simulink model "s_b16a4x32kf"  (R2018a)
settings: Solver=VariableStepDiscrete  StartTime=0.0  StopTime=1000  RelTol=1e-3
undefined symbols (not defined in the file): fft_stages, n_bits_ants, n_bits_xengs
libraries: xbsIndex_r4 x23740, casper_library_misc x48, casper_library_delays x8, xps_library x4, casper_library_scopes x1
(part 48 of 219)

== system s_b16a4x32kf/sys0/xeng/baseline_tap7 ==
  a_del : Inport
  a_ndel : Inport  Port=2
  a_end : Inport  Port=3
  acc_in : Inport  Port=4
  valid_in : Inport  Port=5
  rst : Inport  Port=6
  sync1 : Inport  Port=7
  Constant : xbsIndex_r4/Constant  const=ant_sep * acc_len  gui_display_data_type=Fixed-point  arith_type=Unsigned  n_bits=ant_bits + bit_growth  bin_pt=0  preci_type=Single  exp_width=8  frac_width=24  explicit_period=on  period=1  equ=P=C  opselect=C  inp2=PCIN>>17  opr=+  inp1=P  carry=CIN  dbl_ovrd=off  block_type=constant
      settings: block_version=9.1.01
  Convert : xbsIndex_r4/Convert  gui_display_data_type=Fixed-point  arith_type=Unsigned  n_bits=1  bin_pt=0  float_type=Single  exp_bits=8  fraction_bits=24  quantization=Truncate  overflow=Wrap  en=off  latency=0  pipeline=off  dbl_ovrd=off  block_type=convert
      settings: xl_area=[0, 0, 0, 0, 0, 0, 0]
  Counter : xbsIndex_r4/Counter  cnt_type=Count Limited  cnt_to=n_ants * acc_len - 1  operation=Up  start_count=0  cnt_by_val=1  arith_type=Unsigned  n_bits=ant_bits + bit_growth  bin_pt=0  load_pin=off  rst=on  en=off  explicit_period=off  period=1  use_behavioral_HDL=off  implementation=Fabric  use_rpm=on  dbl_ovrd=off  block_type=counter
      settings: xl_area=[0, 0, 0, 0, 0, 0, 0]  block_version=9.1.01
  Delay{1,3,7..8} (4 alike) : xbsIndex_r4/Delay  rst=off  infoeditControl=Selection of Reset will increase slice count due to use of real FFs and instead of SRLs  en=off  latency=1  reg_retiming=on  dbl_ovrd=off  block_type=delay
      settings: xl_area=[0, 0, 0, 0, 0, 0, 0]  block_version=9.1.01
  Mux : xbsIndex_r4/Mux  inputs=2  en=off  latency=1  precision=Full  arith_type="Signed  (2's comp)"  n_bits=8  bin_pt=2  quantization=Truncate  overflow=Wrap  dbl_ovrd=off  block_type=mux
      settings: xl_area=[0, 0, 0, 0, 0, 0, 0]  block_version=9.1.01
  Relational : xbsIndex_r4/Relational  mode=a<b  op_type=Bool  en=off  latency=0  dbl_ovrd=off  block_type=relational
      settings: xl_area=[0, 0, 0, 0, 0, 0, 0]  block_version=9.1.01
  delay : Subsystem  AncestorBlock=casper_library_delays/delay_bram  mask(delay_bram){DelayLen=acc_len, bram_latency=bram_latency, use_dsp48=off, async=off}
      mask prompts: DelayLen "Delay By:"; bram_latency "BRAM Latency"; use_dsp48 "Use DSP48"; async "asynchronous operation"
      mask help: A delay block that uses BRAM for its storage.
      mask init:
      | delay_bram_init(gcb, ...
      |     'DelayLen', DelayLen, ...
      |     'bram_latency', bram_latency, ...
      |     'use_dsp48', use_dsp48, ...
      |     'async', async);
      mask Help: eval('xlWeb(''http://casper.berkeley.edu/wiki/Delay_bram'')')
  dual_pol_cmac : Subsystem  AncestorBlock=casper_library_correlator/dual_pol_cmac  mask{acc_len=256, n_bits_in=8, bin_pt_in=7, mult_latency=4, add_latency=3, multiplier_implementation=embedded multiplier core}
      mask prompts: acc_len "Number of accumulations"; n_bits_in "Number of bits in"; bin_pt_in "Binary point in"; mult_latency "Multiplier latency"; add_latency "Adder latency"; multiplier_implementation "Multiplier implementation"
      mask init: same as s_b16a4x32kf/sys0/xeng/auto_tap/dual_pol_cmac
      mask TypeOptions multiplier_implementation: behavioral HDL | standard core | embedded multiplier core
  a_del_out : Outport
  a_ndel_out : Outport  Port=2
  a_end_out : Outport  Port=3
  acc_out : Outport  Port=4
  valid_out : Outport  Port=5
  rst_out : Outport  Port=6
  sync_out : Outport  Port=7
  wires:
  delay/1(dout) -> Delay3/1
  Mux/1 -> dual_pol_cmac/2(a2)
  Counter/1 -> Relational/1
  Constant/1 -> Relational/2
  Relational/1 -> Convert/1
  Convert/1 -> Mux/1
  rst/1 -> Delay1/1, Counter/1
  a_del/1 -> delay/1(din)
  dual_pol_cmac/1(acc_out) -> acc_out/1
  acc_in/1 -> dual_pol_cmac/3(acc_in)
  dual_pol_cmac/2(valid_out) -> valid_out/1
  valid_in/1 -> dual_pol_cmac/5(valid_in)
  a_ndel/1 -> Mux/2, Delay7/1
  a_end/1 -> Mux/3, Delay8/1
  Delay3/1 -> a_del_out/1, dual_pol_cmac/1(a1)
  Delay7/1 -> a_ndel_out/1
  Delay8/1 -> a_end_out/1
  Delay1/1 -> rst_out/1, dual_pol_cmac/4(sync)
  sync1/1 -> sync_out/1

== system s_b16a4x32kf/sys0/xeng/baseline_tap8 ==
  a_del : Inport
  a_ndel : Inport  Port=2
  a_end : Inport  Port=3
  acc_in : Inport  Port=4
  valid_in : Inport  Port=5
  rst : Inport  Port=6
  sync1 : Inport  Port=7
  Constant : xbsIndex_r4/Constant  const=ant_sep * acc_len  gui_display_data_type=Fixed-point  arith_type=Unsigned  n_bits=ant_bits + bit_growth  bin_pt=0  preci_type=Single  exp_width=8  frac_width=24  explicit_period=on  period=1  equ=P=C  opselect=C  inp2=PCIN>>17  opr=+  inp1=P  carry=CIN  dbl_ovrd=off  block_type=constant
      settings: block_version=9.1.01
  Convert : xbsIndex_r4/Convert  gui_display_data_type=Fixed-point  arith_type=Unsigned  n_bits=1  bin_pt=0  float_type=Single  exp_bits=8  fraction_bits=24  quantization=Truncate  overflow=Wrap  en=off  latency=0  pipeline=off  dbl_ovrd=off  block_type=convert
      settings: xl_area=[0, 0, 0, 0, 0, 0, 0]
  Counter : xbsIndex_r4/Counter  cnt_type=Count Limited  cnt_to=n_ants * acc_len - 1  operation=Up  start_count=0  cnt_by_val=1  arith_type=Unsigned  n_bits=ant_bits + bit_growth  bin_pt=0  load_pin=off  rst=on  en=off  explicit_period=off  period=1  use_behavioral_HDL=off  implementation=Fabric  use_rpm=on  dbl_ovrd=off  block_type=counter
      settings: xl_area=[0, 0, 0, 0, 0, 0, 0]  block_version=9.1.01
  Delay{1,3,7..8} (4 alike) : xbsIndex_r4/Delay  rst=off  infoeditControl=Selection of Reset will increase slice count due to use of real FFs and instead of SRLs  en=off  latency=1  reg_retiming=on  dbl_ovrd=off  block_type=delay
      settings: xl_area=[0, 0, 0, 0, 0, 0, 0]  block_version=9.1.01
  Mux : xbsIndex_r4/Mux  inputs=2  en=off  latency=1  precision=Full  arith_type="Signed  (2's comp)"  n_bits=8  bin_pt=2  quantization=Truncate  overflow=Wrap  dbl_ovrd=off  block_type=mux
      settings: xl_area=[0, 0, 0, 0, 0, 0, 0]  block_version=9.1.01
  Relational : xbsIndex_r4/Relational  mode=a<b  op_type=Bool  en=off  latency=0  dbl_ovrd=off  block_type=relational
      settings: xl_area=[0, 0, 0, 0, 0, 0, 0]  block_version=9.1.01
  delay : Subsystem  AncestorBlock=casper_library_delays/delay_bram  mask(delay_bram){DelayLen=acc_len, bram_latency=bram_latency, use_dsp48=off, async=off}
      mask prompts: DelayLen "Delay By:"; bram_latency "BRAM Latency"; use_dsp48 "Use DSP48"; async "asynchronous operation"
      mask help: A delay block that uses BRAM for its storage.
      mask init:
      | delay_bram_init(gcb, ...
      |     'DelayLen', DelayLen, ...
      |     'bram_latency', bram_latency, ...
      |     'use_dsp48', use_dsp48, ...
      |     'async', async);
      mask Help: eval('xlWeb(''http://casper.berkeley.edu/wiki/Delay_bram'')')
  dual_pol_cmac : Subsystem  AncestorBlock=casper_library_correlator/dual_pol_cmac  mask{acc_len=256, n_bits_in=8, bin_pt_in=7, mult_latency=4, add_latency=3, multiplier_implementation=embedded multiplier core}
      mask prompts: acc_len "Number of accumulations"; n_bits_in "Number of bits in"; bin_pt_in "Binary point in"; mult_latency "Multiplier latency"; add_latency "Adder latency"; multiplier_implementation "Multiplier implementation"
      mask init: same as s_b16a4x32kf/sys0/xeng/auto_tap/dual_pol_cmac
      mask TypeOptions multiplier_implementation: behavioral HDL | standard core | embedded multiplier core
  a_del_out : Outport
  a_ndel_out : Outport  Port=2
  a_end_out : Outport  Port=3
  acc_out : Outport  Port=4
  valid_out : Outport  Port=5
  rst_out : Outport  Port=6
  sync_out : Outport  Port=7
  wires:
  delay/1(dout) -> Delay3/1
  Mux/1 -> dual_pol_cmac/2(a2)
  Counter/1 -> Relational/1
  Constant/1 -> Relational/2
  Relational/1 -> Convert/1
  Convert/1 -> Mux/1
  rst/1 -> Delay1/1, Counter/1
  a_del/1 -> delay/1(din)
  dual_pol_cmac/1(acc_out) -> acc_out/1
  acc_in/1 -> dual_pol_cmac/3(acc_in)
  dual_pol_cmac/2(valid_out) -> valid_out/1
  valid_in/1 -> dual_pol_cmac/5(valid_in)
  a_ndel/1 -> Mux/2, Delay7/1
  a_end/1 -> Mux/3, Delay8/1
  Delay3/1 -> a_del_out/1, dual_pol_cmac/1(a1)
  Delay7/1 -> a_ndel_out/1
  Delay8/1 -> a_end_out/1
  Delay1/1 -> rst_out/1, dual_pol_cmac/4(sync)
  sync1/1 -> sync_out/1

== system s_b16a4x32kf/sys0/xeng/sample_and_hold1 ==
  sync : Inport
  in : Inport  Port=2
  Constant3 : xbsIndex_r4/Constant  const=period-1  gui_display_data_type=Fixed-point  arith_type=Unsigned  n_bits=ceil(log2(period))  bin_pt=0  preci_type=Single  exp_width=8  frac_width=24  explicit_period=on  period=1  equ=P=C  opselect=C  inp2=PCIN>>17  opr=+  inp1=P  carry=CIN  dbl_ovrd=off  block_type=constant
  Counter4 : xbsIndex_r4/Counter  cnt_type=Free Running  cnt_to=Inf  operation=Up  start_count=0  cnt_by_val=1  arith_type=Unsigned  n_bits=ceil(log2(period))  bin_pt=0  load_pin=off  rst=on  en=off  explicit_period=on  period=1  use_behavioral_HDL=off  implementation=Fabric  use_rpm=on  dbl_ovrd=off  block_type=counter
      settings: xl_area=[0, 0, 0, 0, 0, 0, 0]
  Delay10 : xbsIndex_r4/Delay  rst=off  infoeditControl=Selection of Reset will increase slice count due to use of real FFs and instead of SRLs  en=off  latency=1  reg_retiming=on  dbl_ovrd=off  block_type=delay
      settings: xl_area=[0, 0, 0, 0, 0, 0, 0]
  Logical : xbsIndex_r4/Logical  logical_function=OR  inputs=2  en=off  latency=0  precision=Full  arith_type=Unsigned  n_bits=16  bin_pt=0  align_bp=on  dbl_ovrd=off  block_type=logical
  Register : xbsIndex_r4/Register  init=0  rst=off  en=on  dbl_ovrd=off  block_type=register
  Relational : xbsIndex_r4/Relational  mode=a>=b  op_type=Bool  en=off  latency=0  dbl_ovrd=off  block_type=relational
      settings: xl_area=[0, 0, 0, 0, 0, 0, 0]  block_version=10.1.3
  out : Outport
  wires:
  Relational/1 -> Logical/1
  Constant3/1 -> Relational/2
  Counter4/1 -> Relational/1
  Logical/1 -> Counter4/1, Delay10/1
  sync/1 -> Logical/2
  Register/1 -> out/1
  in/1 -> Register/1
  Delay10/1 -> Register/2

== system s_b16a4x32kf/sys0/xeng/sample_and_hold2 ==
  sync : Inport
  in : Inport  Port=2
  Constant3 : xbsIndex_r4/Constant  const=period-1  gui_display_data_type=Fixed-point  arith_type=Unsigned  n_bits=ceil(log2(period))  bin_pt=0  preci_type=Single  exp_width=8  frac_width=24  explicit_period=on  period=1  equ=P=C  opselect=C  inp2=PCIN>>17  opr=+  inp1=P  carry=CIN  dbl_ovrd=off  block_type=constant
  Counter4 : xbsIndex_r4/Counter  cnt_type=Free Running  cnt_to=Inf  operation=Up  start_count=0  cnt_by_val=1  arith_type=Unsigned  n_bits=ceil(log2(period))  bin_pt=0  load_pin=off  rst=on  en=off  explicit_period=on  period=1  use_behavioral_HDL=off  implementation=Fabric  use_rpm=on  dbl_ovrd=off  block_type=counter
      settings: xl_area=[0, 0, 0, 0, 0, 0, 0]
  Delay10 : xbsIndex_r4/Delay  rst=off  infoeditControl=Selection of Reset will increase slice count due to use of real FFs and instead of SRLs  en=off  latency=1  reg_retiming=on  dbl_ovrd=off  block_type=delay
      settings: xl_area=[0, 0, 0, 0, 0, 0, 0]
  Logical : xbsIndex_r4/Logical  logical_function=OR  inputs=2  en=off  latency=0  precision=Full  arith_type=Unsigned  n_bits=16  bin_pt=0  align_bp=on  dbl_ovrd=off  block_type=logical
  Register : xbsIndex_r4/Register  init=0  rst=off  en=on  dbl_ovrd=off  block_type=register
  Relational : xbsIndex_r4/Relational  mode=a>=b  op_type=Bool  en=off  latency=0  dbl_ovrd=off  block_type=relational
      settings: xl_area=[0, 0, 0, 0, 0, 0, 0]  block_version=10.1.3
  out : Outport
  wires:
  Relational/1 -> Logical/1
  Constant3/1 -> Relational/2
  Counter4/1 -> Relational/1
  Logical/1 -> Counter4/1, Delay10/1
  sync/1 -> Logical/2
  Register/1 -> out/1
  in/1 -> Register/1
  Delay10/1 -> Register/2

== system s_b16a4x32kf/sys0/xeng/sample_and_hold3 ==
  sync : Inport
  in : Inport  Port=2
  Constant3 : xbsIndex_r4/Constant  const=period-1  gui_display_data_type=Fixed-point  arith_type=Unsigned  n_bits=ceil(log2(period))  bin_pt=0  preci_type=Single  exp_width=8  frac_width=24  explicit_period=on  period=1  equ=P=C  opselect=C  inp2=PCIN>>17  opr=+  inp1=P  carry=CIN  dbl_ovrd=off  block_type=constant
  Counter4 : xbsIndex_r4/Counter  cnt_type=Free Running  cnt_to=Inf  operation=Up  start_count=0  cnt_by_val=1  arith_type=Unsigned  n_bits=ceil(log2(period))  bin_pt=0  load_pin=off  rst=on  en=off  explicit_period=on  period=1  use_behavioral_HDL=off  implementation=Fabric  use_rpm=on  dbl_ovrd=off  block_type=counter
      settings: xl_area=[0, 0, 0, 0, 0, 0, 0]
  Delay10 : xbsIndex_r4/Delay  rst=off  infoeditControl=Selection of Reset will increase slice count due to use of real FFs and instead of SRLs  en=off  latency=1  reg_retiming=on  dbl_ovrd=off  block_type=delay
      settings: xl_area=[0, 0, 0, 0, 0, 0, 0]
  Logical : xbsIndex_r4/Logical  logical_function=OR  inputs=2  en=off  latency=0  precision=Full  arith_type=Unsigned  n_bits=16  bin_pt=0  align_bp=on  dbl_ovrd=off  block_type=logical
  Register : xbsIndex_r4/Register  init=0  rst=off  en=on  dbl_ovrd=off  block_type=register
  Relational : xbsIndex_r4/Relational  mode=a>=b  op_type=Bool  en=off  latency=0  dbl_ovrd=off  block_type=relational
      settings: xl_area=[0, 0, 0, 0, 0, 0, 0]  block_version=10.1.3
  out : Outport
  wires:
  Relational/1 -> Logical/1
  Constant3/1 -> Relational/2
  Counter4/1 -> Relational/1
  Logical/1 -> Counter4/1, Delay10/1
  sync/1 -> Logical/2
  Register/1 -> out/1
  in/1 -> Register/1
  Delay10/1 -> Register/2

== system s_b16a4x32kf/sys0/xeng/xeng_descramble ==
  note: x_cast is necessary to correct for BRAM
      | readout order
  note: This bit of logic
      | ensures that we only send out
      | a sync if one was received
      | (and then align it with the start of a read)
  acc : Inport
  valid : Inport  Port=2
  sync : Inport  Port=3
  win_valid : Inport  Port=4
  Constant2 : xbsIndex_r4/Constant  const=0  gui_display_data_type=Fixed-point  arith_type=Boolean  n_bits=elements_bits + 1  bin_pt=0  preci_type=Single  exp_width=8  frac_width=24  explicit_period=on  period=1  equ=P=C  opselect=C  inp2=PCIN>>17  opr=+  inp1=P  carry=CIN  dbl_ovrd=off  block_type=constant
      settings: block_version=9.2.01
  Constant3 : xbsIndex_r4/Constant  const=0  gui_display_data_type=Fixed-point  arith_type=Unsigned  n_bits=n_bits_in/demux_factor  bin_pt=0  preci_type=Single  exp_width=8  frac_width=24  explicit_period=on  period=1  equ=P=C  opselect=C  inp2=PCIN>>17  opr=+  inp1=P  carry=CIN  dbl_ovrd=off  block_type=constant
      settings: block_version=9.2.01
  Delay{1..4} (4 alike) : xbsIndex_r4/Delay  rst=off  infoeditControl=Selection of Reset will increase slice count due to use of real FFs and instead of SRLs  en=off  latency=1  reg_retiming=off  dbl_ovrd=off  block_type=delay
      settings: xl_area=[0, 0, 0, 0, 0, 0, 0]  block_version=9.2.01
  Delay5 : xbsIndex_r4/Delay  rst=off  infoeditControl=Selection of Reset will increase slice count due to use of real FFs and instead of SRLs  en=off  latency=2  reg_retiming=off  dbl_ovrd=off  block_type=delay
      settings: xl_area=[0, 0, 0, 0, 0, 0, 0]  block_version=9.2.01
  Delay6 : xbsIndex_r4/Delay  rst=off  infoeditControl=Selection of Reset will increase slice count due to use of real FFs and instead of SRLs  en=off  latency=2  reg_retiming=off  dbl_ovrd=off  block_type=delay
      settings: xl_area=[0, 0, 0, 0, 0, 0, 0]  block_version=9.2.01
  Dual Port RAM : xbsIndex_r4/Dual Port RAM  depth=(num_elements+1)*demux_factor  initVector=[1:36*8]  distributed_mem=Block RAM  init_a=0  init_b=0  rst_a=off  rst_b=off  en_a=off  en_b=off  latency=1  write_mode_A=No Read On Write  write_mode_B=No Read On Write  optimize=Area  dbl_ovrd=off  block_type=dpram
      settings: xl_area=[0, 0, 0, 0, 0, 0, 0]  block_version=9.2.01
  Gateway Out{1..11,17,19..20} (14 alike) : xbsIndex_r4/Gateway Out  inherit_from_input=off  hdl_port=off  rows=1  columns=1  UseAsDAC=off  DACChannel='1'  interface=None  automatic_assignment=on  address_offset=hex2dec('00')  intf_name=''  intf_description=''  timing_constraint=None  locs_specified=off  LOCs={}  io_standard={}  block_type=gatewayout
      settings: infoedit="Gateway out block.  Converts Xilinx fixed point inputs into ouputs of type Simulink integer, double, or fixed point.<P><P>Hardware notes:  In hardware these blocks become top level output ports or are discarded, depending on how they are configured."  xl_area=[0, 0, 0, 0, 0, 0, 0]  block_version=10.1.3
  Logical : xbsIndex_r4/Logical  logical_function=AND  inputs=2  en=off  latency=1  precision=Full  arith_type=Unsigned  n_bits=16  bin_pt=0  align_bp=on  dbl_ovrd=off  block_type=logical
  Register : xbsIndex_r4/Register  init=0  rst=on  en=on  dbl_ovrd=off  block_type=register
  Scope1 : Scope  NumInputPorts=8
  Scope6 : Scope  NumInputPorts=6
  Terminator1 : Terminator
  read_ctrl : Subsystem
  write_ctrl : Subsystem
  x_cast : Subsystem  mask{n_bits_in=n_bits_xeng_out, n_bits_out=n_bits_in/8, fix_pnt_pos=(n_bits-1)*2, demux_factor=demux_factor}
      mask prompts: n_bits_in "Number of bits (input)"; n_bits_out "Number of bits (output)"; fix_pnt_pos "Fixed point position"; demux_factor "Demux Factor"
      mask init: same as s_b16a4x32kf/sys0/x_cast
      settings: AttributesFormatString=25 -> 32, demux 1.
  acc_out : Outport
  valid_out : Outport  Port=2
  sync_out : Outport  Port=3
  wires:
  x_cast/1(out) -> Delay4/1, Dual Port RAM/5
  Delay6/1 -> Gateway Out6/1
  Delay5/1 -> Gateway Out8/1
  [sync_in] -> Register/3
  [sync_in] -> Register/1
  [sync_in] -> Gateway Out5/1
  [valid_out] -> Gateway Out7/1
  [valid_out] -> Delay1/1
  read_ctrl/2(enable) -> [valid_out]
  [start_read] -> Gateway Out4/1
  [start_read] -> Register/2
  [start_read] -> Logical/1
  [start_read] -> read_ctrl/1(start)
  write_ctrl/1(start_readout) -> [start_read]
  win_valid/1 -> Delay5/1, write_ctrl/4(window_valid)
  Register/1 -> Logical/2
  Logical/1 -> Gateway Out3/1, sync_out/1
  Delay4/1 -> Gateway Out17/1
  Delay3/1 -> Gateway Out19/1
  Delay2/1 -> Gateway Out20/1
  Gateway Out10/1 -> Scope1/7
  Gateway Out9/1 -> Scope1/6
  Gateway Out7/1 -> Scope1/5
  Gateway Out4/1 -> Scope1/4
  Gateway Out5/1 -> Scope1/1
  Gateway Out6/1 -> Scope1/2
  Gateway Out8/1 -> Scope1/3
  Gateway Out3/1 -> Scope6/6
  Gateway Out2/1 -> Scope6/5
  Gateway Out1/1 -> Scope6/4
  Gateway Out17/1 -> Scope6/1
  Gateway Out19/1 -> Scope6/2
  Gateway Out20/1 -> Scope6/3
  Dual Port RAM/2 -> Terminator1/1
  acc/1 -> write_ctrl/2(data_in)
  write_ctrl/3(data_out) -> x_cast/1(in)
  Constant3/1 -> Dual Port RAM/2
  write_ctrl/4(enable) -> Delay3/1, Dual Port RAM/6, Gateway Out10/1
  Constant2/1 -> Dual Port RAM/3
  Delay1/1 -> Gateway Out2/1, valid_out/1
  Dual Port RAM/1 -> Gateway Out1/1, acc_out/1
  read_ctrl/1(read_addr) -> Gateway Out9/1, Delay2/1, Dual Port RAM/1
  write_ctrl/2(write_addr) -> Dual Port RAM/4, Gateway Out11/1
  sync/1 -> [sync_in], write_ctrl/1(sync)
  valid/1 -> Delay6/1, write_ctrl/3(xeng_valid)
  Gateway Out11/1 -> Scope1/8

== system s_b16a4x32kf/sys0/xeng_pack_out/edge_detect ==
  in : Inport
  Delay : xbsIndex_r4/Delay  rst=off  infoeditControl=Selection of Reset will increase slice count due to use of real FFs and instead of SRLs  en=off  latency=1  reg_retiming=on  dbl_ovrd=off  block_type=delay
      settings: xl_area=[0, 0, 0, 0, 0, 0, 0]
  Inverter : xbsIndex_r4/Inverter  en=off  latency=0  dbl_ovrd=off  block_type=inv
      settings: xl_area=[0, 0, 0, 0, 0, 0, 0]
  edge_op : xbsIndex_r4/Logical  logical_function=NOR  inputs=2  en=off  latency=0  precision=Full  arith_type=Unsigned  n_bits=8  bin_pt=2  align_bp=on  dbl_ovrd=off  block_type=logical
      settings: xl_area=[0, 0, 0, 0, 0, 0, 0]
  out : Outport
  wires:
  Inverter/1 -> edge_op/1
  edge_op/1 -> out/1
  in/1 -> Inverter/1, Delay/1
  Delay/1 -> edge_op/2

== system s_b16a4x32kf/sys0/xeng_pack_out/edge_detect1 ==
  in : Inport
  Delay : xbsIndex_r4/Delay  rst=off  infoeditControl=Selection of Reset will increase slice count due to use of real FFs and instead of SRLs  en=off  latency=1  reg_retiming=on  dbl_ovrd=off  block_type=delay
      settings: xl_area=[0, 0, 0, 0, 0, 0, 0]
  Inverter : xbsIndex_r4/Inverter  en=off  latency=0  dbl_ovrd=off  block_type=inv
      settings: xl_area=[0, 0, 0, 0, 0, 0, 0]
  edge_op : xbsIndex_r4/Logical  logical_function=NOR  inputs=2  en=off  latency=0  precision=Full  arith_type=Unsigned  n_bits=8  bin_pt=2  align_bp=on  dbl_ovrd=off  block_type=logical
      settings: xl_area=[0, 0, 0, 0, 0, 0, 0]
  out : Outport
  wires:
  Delay/1 -> edge_op/2
  in/1 -> Delay/1, Inverter/1
  edge_op/1 -> out/1
  Inverter/1 -> edge_op/1

== system s_b16a4x32kf/sys0/xeng_pack_out/edge_detect2 ==
  in : Inport
  Delay : xbsIndex_r4/Delay  rst=off  infoeditControl=Selection of Reset will increase slice count due to use of real FFs and instead of SRLs  en=off  latency=1  reg_retiming=on  dbl_ovrd=off  block_type=delay
      settings: xl_area=[0, 0, 0, 0, 0, 0, 0]
  Inverter : xbsIndex_r4/Inverter  en=off  latency=0  dbl_ovrd=off  block_type=inv
      settings: xl_area=[0, 0, 0, 0, 0, 0, 0]
  edge_op : xbsIndex_r4/Logical  logical_function=NOR  inputs=2  en=off  latency=0  precision=Full  arith_type=Unsigned  n_bits=8  bin_pt=2  align_bp=on  dbl_ovrd=off  block_type=logical
      settings: xl_area=[0, 0, 0, 0, 0, 0, 0]
  out : Outport
  wires:
  Inverter/1 -> edge_op/1
  edge_op/1 -> out/1
  in/1 -> Inverter/1, Delay/1
  Delay/1 -> edge_op/2

== system s_b16a4x32kf/sys0/xeng_pack_out/edge_detect3 ==
  in : Inport
  Delay : xbsIndex_r4/Delay  rst=off  infoeditControl=Selection of Reset will increase slice count due to use of real FFs and instead of SRLs  en=off  latency=1  reg_retiming=on  dbl_ovrd=off  block_type=delay
      settings: xl_area=[0, 0, 0, 0, 0, 0, 0]
  Inverter : xbsIndex_r4/Inverter  en=off  latency=0  dbl_ovrd=off  block_type=inv
      settings: xl_area=[0, 0, 0, 0, 0, 0, 0]
  edge_op : xbsIndex_r4/Logical  logical_function=NOR  inputs=2  en=off  latency=0  precision=Full  arith_type=Unsigned  n_bits=8  bin_pt=2  align_bp=on  dbl_ovrd=off  block_type=logical
      settings: xl_area=[0, 0, 0, 0, 0, 0, 0]
  out : Outport
  wires:
  Delay/1 -> edge_op/2
  in/1 -> Delay/1, Inverter/1
  edge_op/1 -> out/1
  Inverter/1 -> edge_op/1

== system s_b16a4x32kf/sys0/xeng_pack_out/edge_detect7 ==
  in : Inport
  Delay : xbsIndex_r4/Delay  rst=off  infoeditControl=Selection of Reset will increase slice count due to use of real FFs and instead of SRLs  en=off  latency=1  reg_retiming=on  dbl_ovrd=off  block_type=delay
      settings: xl_area=[0, 0, 0, 0, 0, 0, 0]
  Inverter : xbsIndex_r4/Inverter  en=off  latency=0  dbl_ovrd=off  block_type=inv
      settings: xl_area=[0, 0, 0, 0, 0, 0, 0]
  edge_op : xbsIndex_r4/Logical  logical_function=NOR  inputs=2  en=off  latency=0  precision=Full  arith_type=Unsigned  n_bits=8  bin_pt=2  align_bp=on  dbl_ovrd=off  block_type=logical
      settings: xl_area=[0, 0, 0, 0, 0, 0, 0]
  out : Outport
  wires:
  Delay/1 -> edge_op/2
  in/1 -> Delay/1, Inverter/1
  edge_op/1 -> out/1
  Inverter/1 -> edge_op/1

== system s_b16a4x32kf/sys0/xeng_pack_out/pack_xeng ==
  note: eof ON the last valid data.
  note: SPEAD header
  note: magic number - 0x53
  note: spead version
  note: item id width in bytes
  note: heap addr width in bytes
  note: <reserved>
  note: num item pointers -
      | after this header
  data256_ready : Inport
  data256_valid : Inport  Port=2
  data256 : Inport  Port=3
  hdr_heap_id : Inport  Port=4
  hdr_heap_size : Inport  Port=5
  hdr_heap_offset : Inport  Port=6
  hdr_pkt_len_words : Inport  Port=7
  hdr5_0x1600_DIR : Inport  Port=8
  hdr6_0x4103_DIR : Inport  Port=9
  hdr8_0x1800 : Inport  Port=10
  AddSub1 : xbsIndex_r4/AddSub  mode=Subtraction  use_carryin=off  use_carryout=off  en=off  latency=0  precision=Full  arith_type=Unsigned  n_bits=16  bin_pt=14  quantization=Truncate  overflow=Wrap  use_behavioral_HDL=off  hw_selection=Fabric  pipelined=off  dbl_ovrd=off  block_type=addsub
  Assert17 : xbsIndex_r4/Assert  assert_type=on  type_source=Explicitly  gui_display_data_type=Fixed-point  arith_type=Unsigned  n_bits=64  bin_pt=0  preci_type=Single  exp_width=8  frac_width=24  assert_rate=off  rate_source=Explicitly  period=1  output_port=on  block_type=assert
  Assert18 : xbsIndex_r4/Assert  assert_type=on  type_source=Explicitly  gui_display_data_type=Fixed-point  arith_type=Unsigned  n_bits=256  bin_pt=0  preci_type=Single  exp_width=8  frac_width=24  assert_rate=off  rate_source=Explicitly  period=1  output_port=on  block_type=assert
  Assert5 : xbsIndex_r4/Assert  assert_type=on  type_source=Explicitly  gui_display_data_type=Fixed-point  arith_type=Boolean  n_bits=64  bin_pt=0  preci_type=Single  exp_width=8  frac_width=24  assert_rate=off  rate_source=Explicitly  period=1  output_port=on  block_type=assert
      settings: block_version=10.1.3
  Assert6 : xbsIndex_r4/Assert  assert_type=on  type_source=Explicitly  gui_display_data_type=Fixed-point  arith_type=Unsigned  n_bits=256  bin_pt=0  preci_type=Single  exp_width=8  frac_width=24  assert_rate=off  rate_source=Explicitly  period=1  output_port=on  block_type=assert
      settings: block_version=10.1.3
  Assert7 : xbsIndex_r4/Assert  assert_type=on  type_source=Explicitly  gui_display_data_type=Boolean  arith_type=Boolean  n_bits=64  bin_pt=0  preci_type=Single  exp_width=8  frac_width=24  assert_rate=off  rate_source=Explicitly  period=1  output_port=on  block_type=assert
      settings: block_version=10.1.3
  Concat : xbsIndex_r4/Concat  num_inputs=6  dbl_ovrd=off  block_type=concat
      settings: block_version=10.1.3
  Concat1 : xbsIndex_r4/Concat  num_inputs=4  dbl_ovrd=off  block_type=concat
      settings: block_version=10.1.3
  Concat3 : xbsIndex_r4/Concat  num_inputs=4  dbl_ovrd=off  block_type=concat
      settings: block_version=10.1.3
  Constant3 : xbsIndex_r4/Constant  const=83  gui_display_data_type=Fixed-point  arith_type=Unsigned  n_bits=8  bin_pt=0  preci_type=Single  exp_width=8  frac_width=24  explicit_period=on  period=1  equ=P=C  opselect=C  inp2=PCIN>>17  opr=+  inp1=P  carry=CIN  dbl_ovrd=off  block_type=constant
  Constant4 : xbsIndex_r4/Constant  const=spead_version  gui_display_data_type=Fixed-point  arith_type=Unsigned  n_bits=8  bin_pt=0  preci_type=Single  exp_width=8  frac_width=24  explicit_period=on  period=1  equ=P=C  opselect=C  inp2=PCIN>>17  opr=+  inp1=P  carry=CIN  dbl_ovrd=off  block_type=constant
  Constant7 : xbsIndex_r4/Constant  const=0  gui_display_data_type=Fixed-point  arith_type=Unsigned  n_bits=16  bin_pt=0  preci_type=Single  exp_width=8  frac_width=24  explicit_period=on  period=1  equ=P=C  opselect=C  inp2=PCIN>>17  opr=+  inp1=P  carry=CIN  dbl_ovrd=off  block_type=constant
  Logical5 : xbsIndex_r4/Logical  logical_function=AND  inputs=2  en=off  latency=0  precision=Full  arith_type=Unsigned  n_bits=8  bin_pt=2  align_bp=on  dbl_ovrd=off  block_type=logical
      settings: xl_area=[0, 0, 0, 0, 0, 0, 0]
  Logical6 : xbsIndex_r4/Logical  logical_function=OR  inputs=2  en=off  latency=0  precision=Full  arith_type=Unsigned  n_bits=8  bin_pt=2  align_bp=on  dbl_ovrd=off  block_type=logical
      settings: xl_area=[0, 0, 0, 0, 0, 0, 0]
  Logical7 : xbsIndex_r4/Logical  logical_function=OR  inputs=2  en=off  latency=1  precision=Full  arith_type=Unsigned  n_bits=8  bin_pt=2  align_bp=on  dbl_ovrd=off  block_type=logical
      settings: xl_area=[0, 0, 0, 0, 0, 0, 0]
  Logical8 : xbsIndex_r4/Logical  logical_function=OR  inputs=2  en=off  latency=0  precision=Full  arith_type=Unsigned  n_bits=8  bin_pt=2  align_bp=on  dbl_ovrd=off  block_type=logical
      settings: xl_area=[0, 0, 0, 0, 0, 0, 0]
  Register2 : xbsIndex_r4/Register  init=0  rst=on  en=on  dbl_ovrd=off  block_type=register
  Relational3 : xbsIndex_r4/Relational  mode=a=b  op_type=Bool  en=off  latency=0  dbl_ovrd=off  block_type=relational
      settings: xl_area=[0, 0, 0, 0, 0, 0, 0]  block_version=10.1.3
  assert_data2 : xbsIndex_r4/Assert  assert_type=on  type_source=Explicitly  gui_display_data_type=Fixed-point  arith_type=Unsigned  n_bits=256  bin_pt=0  preci_type=Single  exp_width=8  frac_width=24  assert_rate=off  rate_source=Explicitly  period=1  output_port=on  block_type=assert
  assert_data3 : xbsIndex_r4/Assert  assert_type=on  type_source=Explicitly  gui_display_data_type=Fixed-point  arith_type=Unsigned  n_bits=256  bin_pt=0  preci_type=Single  exp_width=8  frac_width=24  assert_rate=off  rate_source=Explicitly  period=1  output_port=on  block_type=assert
  data_ctr1 : xbsIndex_r4/Counter  cnt_type=Free Running  cnt_to=4  operation=Up  start_count=0  cnt_by_val=1  arith_type=Unsigned  n_bits=max_pkt_len_bits + 1  bin_pt=0  load_pin=off  rst=on  en=on  explicit_period=on  period=1  use_behavioral_HDL=off  implementation=Fabric  use_rpm=on  dbl_ovrd=off  block_type=counter
      settings: xl_area=[0, 0, 0, 0, 0, 0, 0]
  delay_data{6,9..10,13,15,17..18,20} (8 alike) : xbsIndex_r4/Delay  rst=off  infoeditControl=Selection of Reset will increase slice count due to use of real FFs and instead of SRLs  en=off  latency=1  reg_retiming=on  dbl_ovrd=off  block_type=delay
      settings: block_version=11.4
  delay_data12 : xbsIndex_r4/Delay  rst=off  infoeditControl=Selection of Reset will increase slice count due to use of real FFs and instead of SRLs  en=off  latency=2  reg_retiming=on  dbl_ovrd=off  block_type=delay
      settings: infoedit=Hardware notes: A delay line is a chain, each link of which is an SRL16 or SRL32 followed by a flip-flop.  block_version=11.4
  delay_data5 : xbsIndex_r4/Delay  rst=off  infoeditControl=Selection of Reset will increase slice count due to use of real FFs and instead of SRLs  en=off  latency=2  reg_retiming=on  dbl_ovrd=off  block_type=delay
      settings: infoedit=Hardware notes: A delay line is a chain, each link of which is an SRL16 or SRL32 followed by a flip-flop.  block_version=11.4
  delay_data7 : xbsIndex_r4/Delay  rst=off  infoeditControl=Selection of Reset will increase slice count due to use of real FFs and instead of SRLs  en=off  latency=2  reg_retiming=on  dbl_ovrd=off  block_type=delay
      settings: infoedit=Hardware notes: A delay line is a chain, each link of which is an SRL16 or SRL32 followed by a flip-flop.  block_version=11.4
  hdra_{1..6,8} (7 alike) : xbsIndex_r4/Assert  assert_type=on  type_source=Explicitly  gui_display_data_type=Fixed-point  arith_type=Unsigned  n_bits=spead_lsw  bin_pt=0  preci_type=Single  exp_width=8  frac_width=24  assert_rate=off  rate_source=Explicitly  period=1  output_port=on  block_type=assert
  header_4cast4 : xbsIndex_r4/Convert  gui_display_data_type=Fixed-point  arith_type=Unsigned  n_bits=spead_lsw - 5  bin_pt=0  float_type=Single  exp_bits=8  fraction_bits=24  quantization=Truncate  overflow=Wrap  en=off  latency=1  pipeline=on  dbl_ovrd=off  block_type=convert
  header_4cat4 : xbsIndex_r4/Concat  num_inputs=2  dbl_ovrd=off  block_type=concat
  header_4const2 : xbsIndex_r4/Constant  const=0  gui_display_data_type=Fixed-point  arith_type=Unsigned  n_bits=spead_lsw  bin_pt=0  preci_type=Single  exp_width=8  frac_width=24  explicit_period=on  period=1  equ=P=C  opselect=C  inp2=PCIN>>17  opr=+  inp1=P  carry=CIN  dbl_ovrd=off  block_type=constant
  header_4const4 : xbsIndex_r4/Constant  const=0  gui_display_data_type=Fixed-point  arith_type=Unsigned  n_bits=5  bin_pt=0  preci_type=Single  exp_width=8  frac_width=24  explicit_period=on  period=1  equ=P=C  opselect=C  inp2=PCIN>>17  opr=+  inp1=P  carry=CIN  dbl_ovrd=off  block_type=constant
  header_assert{1..6,8} (7 alike) : xbsIndex_r4/Assert  assert_type=on  type_source=Explicitly  gui_display_data_type=Fixed-point  arith_type=Unsigned  n_bits=spead_msw  bin_pt=0  preci_type=Single  exp_width=8  frac_width=24  assert_rate=off  rate_source=Explicitly  period=1  output_port=on  block_type=assert
  header_cat{1..6,8} (7 alike) : xbsIndex_r4/Concat  num_inputs=2  dbl_ovrd=off  block_type=concat
  header_const1 : xbsIndex_r4/Constant  const=32769  gui_display_data_type=Fixed-point  arith_type=Unsigned  n_bits=spead_msw - spead_lsw  bin_pt=0  preci_type=Single  exp_width=8  frac_width=24  explicit_period=off  period=1  equ=P=C  opselect=C  inp2=PCIN>>17  opr=+  inp1=P  carry=CIN  dbl_ovrd=off  block_type=constant
  header_const2 : xbsIndex_r4/Constant  const=32770  gui_display_data_type=Fixed-point  arith_type=Unsigned  n_bits=spead_msw - spead_lsw  bin_pt=0  preci_type=Single  exp_width=8  frac_width=24  explicit_period=off  period=1  equ=P=C  opselect=C  inp2=PCIN>>17  opr=+  inp1=P  carry=CIN  dbl_ovrd=off  block_type=constant
  header_const3 : xbsIndex_r4/Constant  const=32771  gui_display_data_type=Fixed-point  arith_type=Unsigned  n_bits=spead_msw - spead_lsw  bin_pt=0  preci_type=Single  exp_width=8  frac_width=24  explicit_period=off  period=1  equ=P=C  opselect=C  inp2=PCIN>>17  opr=+  inp1=P  carry=CIN  dbl_ovrd=off  block_type=constant
  header_const4 : xbsIndex_r4/Constant  const=32772  gui_display_data_type=Fixed-point  arith_type=Unsigned  n_bits=spead_msw - spead_lsw  bin_pt=0  preci_type=Single  exp_width=8  frac_width=24  explicit_period=off  period=1  equ=P=C  opselect=C  inp2=PCIN>>17  opr=+  inp1=P  carry=CIN  dbl_ovrd=off  block_type=constant
  header_const5 : xbsIndex_r4/Constant  const=38400  gui_display_data_type=Fixed-point  arith_type=Unsigned  n_bits=spead_msw - spead_lsw  bin_pt=0  preci_type=Single  exp_width=8  frac_width=24  explicit_period=off  period=1  equ=P=C  opselect=C  inp2=PCIN>>17  opr=+  inp1=P  carry=CIN  dbl_ovrd=off  block_type=constant
  header_const6 : xbsIndex_r4/Constant  const=49411  gui_display_data_type=Fixed-point  arith_type=Unsigned  n_bits=spead_msw - spead_lsw  bin_pt=0  preci_type=Single  exp_width=8  frac_width=24  explicit_period=off  period=1  equ=P=C  opselect=C  inp2=PCIN>>17  opr=+  inp1=P  carry=CIN  dbl_ovrd=off  block_type=constant
  header_const8 : xbsIndex_r4/Constant  const=6144  gui_display_data_type=Fixed-point  arith_type=Unsigned  n_bits=spead_msw - spead_lsw  bin_pt=0  preci_type=Single  exp_width=8  frac_width=24  explicit_period=off  period=1  equ=P=C  opselect=C  inp2=PCIN>>17  opr=+  inp1=P  carry=CIN  dbl_ovrd=off  block_type=constant
  heap_addr_width : xbsIndex_r4/Constant  const=spead_lsw/8  gui_display_data_type=Fixed-point  arith_type=Unsigned  n_bits=8  bin_pt=0  preci_type=Single  exp_width=8  frac_width=24  explicit_period=on  period=1  equ=P=C  opselect=C  inp2=PCIN>>17  opr=+  inp1=P  carry=CIN  dbl_ovrd=off  block_type=constant
  item_id_width : xbsIndex_r4/Constant  const=(spead_msw-spead_lsw)/8  gui_display_data_type=Fixed-point  arith_type=Unsigned  n_bits=8  bin_pt=0  preci_type=Single  exp_width=8  frac_width=24  explicit_period=on  period=1  equ=P=C  opselect=C  inp2=PCIN>>17  opr=+  inp1=P  carry=CIN  dbl_ovrd=off  block_type=constant
  mainmux1 : xbsIndex_r4/Mux  inputs=2  en=off  latency=1  precision=Full  arith_type="Signed  (2's comp)"  n_bits=8  bin_pt=2  quantization=Truncate  overflow=Wrap  dbl_ovrd=off  block_type=mux
      settings: xl_area=[0, 0, 0, 0, 0, 0, 0]
  mainmux2 : xbsIndex_r4/Mux  inputs=2  en=off  latency=1  precision=Full  arith_type="Signed  (2's comp)"  n_bits=8  bin_pt=2  quantization=Truncate  overflow=Wrap  dbl_ovrd=off  block_type=mux
      settings: xl_area=[0, 0, 0, 0, 0, 0, 0]
  num_item_pts : xbsIndex_r4/Constant  const=7  gui_display_data_type=Fixed-point  arith_type=Unsigned  n_bits=16  bin_pt=0  preci_type=Single  exp_width=8  frac_width=24  explicit_period=on  period=1  equ=P=C  opselect=C  inp2=PCIN>>17  opr=+  inp1=P  carry=CIN  dbl_ovrd=off  block_type=constant
  only_one1 : xbsIndex_r4/Constant  const=1  gui_display_data_type=Fixed-point  arith_type=Unsigned  n_bits=1  bin_pt=0  preci_type=Single  exp_width=8  frac_width=24  explicit_period=on  period=1  equ=P=C  opselect=C  inp2=PCIN>>17  opr=+  inp1=P  carry=CIN  dbl_ovrd=off  block_type=constant
  data_out : Outport
  valid_out : Outport  Port=2
  eof : Outport  Port=3
  data_overflow : Outport  Port=4
  wires:
  [out_data] -> Assert18/1
  [out_valid] -> valid_out/1
  [out_overflow] -> data_overflow/1
  [out_done] -> eof/1
  Logical8/1 -> [out_done]  "out_done"
  delay_data20/1 -> [out_overflow], Logical8/2  "out_overflow"
  delay_data18/1 -> delay_data20/1
  Logical5/1 -> delay_data18/1  "overflow"
  Register2/1 -> Logical5/1  "busy"
  delay_data17/1 -> Logical8/1
  delay_data15/1 -> delay_data17/1
  Relational3/1 -> delay_data15/1, Register2/2  "done"
  AddSub1/1 -> Relational3/2
  only_one1/1 -> AddSub1/2
  [hdr_4] -> AddSub1/1
  data_ctr1/1 -> Relational3/1  "data_ctr"
  [in_data256] -> delay_data12/1
  delay_data12/1 -> delay_data13/1
  delay_data9/1 -> [out_valid]  "out_valid"
  Logical7/1 -> delay_data9/1
  [header1] -> mainmux2/3
  [header0] -> mainmux2/2
  delay_data7/1 -> Logical6/2, mainmux2/1
  mainmux1/1 -> [out_data]  "out_data"
  delay_data13/1 -> mainmux1/2
  mainmux2/1 -> mainmux1/3
  delay_data10/1 -> mainmux1/1
  delay_data6/1 -> Logical6/1
  Logical6/1 -> Logical7/1, data_ctr1/1, delay_data10/1  "wr_hdr"
  [in_ready] -> delay_data6/1, delay_data7/1, Register2/1, Register2/3, Logical5/2  "in_rdy"
  delay_data5/1 -> Logical7/2, data_ctr1/2  "wr_data"
  [in_valid] -> delay_data5/1
  assert_data3/1 -> [header1]
  Concat3/1 -> assert_data3/1
  assert_data2/1 -> [header0]
  Concat1/1 -> assert_data2/1
  header_cat8/1 -> header_assert8/1
  [hdr_8] -> header_cat8/2
  header_const8/1 -> header_cat8/1  "spid8"
  hdra_8/1 -> [hdr_8]  "hdr8_0x4300"
  hdr8_0x1800/1 -> hdra_8/1
  header_assert8/1 -> Concat3/4
  header_assert6/1 -> Concat3/3
  header_cat6/1 -> header_assert6/1
  [hdr_6] -> header_cat6/2
  header_const6/1 -> header_cat6/1  "spid6"
  hdra_6/1 -> [hdr_6]  "hdr6_0x4101_DIR"
  hdr6_0x4103_DIR/1 -> hdra_6/1
  header_assert5/1 -> Concat3/2
  header_cat5/1 -> header_assert5/1
  [hdr_5] -> header_cat5/2
  header_const5/1 -> header_cat5/1  "spid5"
  hdra_5/1 -> [hdr_5]  "hdr5_0x1600_DIR"
  hdr5_0x1600_DIR/1 -> hdra_5/1
  header_assert4/1 -> Concat3/1
  header_cat4/1 -> header_assert4/1
  header_4cat4/1 -> header_cat4/2
  header_4const4/1 -> header_4cat4/2
  header_4cast4/1 -> header_4cat4/1
  [hdr_4] -> header_4cast4/1
  header_const4/1 -> header_cat4/1  "spid4"
  hdra_4/1 -> [hdr_4]  "hdr_pkt_len_words"
  hdr_pkt_len_words/1 -> hdra_4/1
  header_assert3/1 -> Concat1/4
  header_cat3/1 -> header_assert3/1
  [hdr_3] -> header_cat3/2
  header_const3/1 -> header_cat3/1  "spid3"
  hdra_3/1 -> [hdr_3]  "hdr_heap_offset"
  hdr_heap_offset/1 -> hdra_3/1
  header_assert2/1 -> Concat1/3
  header_cat2/1 -> header_assert2/1
  [hdr_2] -> header_cat2/2
  header_const2/1 -> header_cat2/1  "spid2"
  hdra_2/1 -> [hdr_2]  "hdr_heap_size"
  hdr_heap_size/1 -> hdra_2/1
  header_assert1/1 -> Concat1/2
  header_cat1/1 -> header_assert1/1
  [hdr_1] -> header_cat1/2
  header_const1/1 -> header_cat1/1  "spid1"
  hdra_1/1 -> [hdr_1]  "hdr_heap_id"
  hdr_heap_id/1 -> hdra_1/1
  num_item_pts/1 -> Concat/6
  Assert18/1 -> data_out/1
  Assert17/1 -> Concat1/1
  Assert7/1 -> [in_valid]  "data64_valid"
  data256_valid/1 -> Assert7/1
  data256_ready/1 -> Assert5/1
  Assert5/1 -> [in_ready]  "data64_rdy"
  Assert6/1 -> [in_data256]  "data64"
  data256/1 -> Assert6/1
  Constant7/1 -> Concat/5
  heap_addr_width/1 -> Concat/4
  item_id_width/1 -> Concat/3
  Constant4/1 -> Concat/2
  Constant3/1 -> Concat/1
  Concat/1 -> Assert17/1  "spd_hdr"

== system s_b16a4x32kf/sys0/xeng_pack_out/status ==
  out_pkt_cnt : Inport
  out_align_err_cnt : Inport  Port=2
  out_overflow_err_cnt : Inport  Port=3
  assert_align_err_cnt : xbsIndex_r4/Assert  assert_type=on  type_source=Explicitly  gui_display_data_type=Fixed-point  arith_type=Unsigned  n_bits=8  bin_pt=0  preci_type=Single  exp_width=8  frac_width=24  assert_rate=off  rate_source=Explicitly  period=1  output_port=on  block_type=assert
  assert_overflow_err_cnt : xbsIndex_r4/Assert  assert_type=on  type_source=Explicitly  gui_display_data_type=Fixed-point  arith_type=Unsigned  n_bits=8  bin_pt=0  preci_type=Single  exp_width=8  frac_width=24  assert_rate=off  rate_source=Explicitly  period=1  output_port=on  block_type=assert
  assert_pkt_cnt : xbsIndex_r4/Assert  assert_type=on  type_source=Explicitly  gui_display_data_type=Fixed-point  arith_type=Unsigned  n_bits=16  bin_pt=0  preci_type=Single  exp_width=8  frac_width=24  assert_rate=off  rate_source=Explicitly  period=1  output_port=on  block_type=assert
  cast_gw : xbsIndex_r4/Convert  gui_display_data_type=Fixed-point  arith_type=Unsigned  n_bits=32  bin_pt=0  float_type=Single  exp_bits=8  fraction_bits=24  quantization=Truncate  overflow=Wrap  en=off  latency=1  pipeline=off  dbl_ovrd=off  block_type=convert
  concatenate : xbsIndex_r4/Concat  num_inputs=3  dbl_ovrd=off  block_type=concat
  io_delay : xbsIndex_r4/Delay  rst=off  infoeditControl=Selection of Reset will increase slice count due to use of real FFs and instead of SRLs  en=off  latency=1  reg_retiming=on  dbl_ovrd=off  block_type=delay
  reint1 : xbsIndex_r4/Reinterpret  force_arith_type=on  arith_type=Unsigned  force_bin_pt=on  bin_pt=0  block_type=reinterpret
  reint2 : xbsIndex_r4/Reinterpret  force_arith_type=on  arith_type=Unsigned  force_bin_pt=on  bin_pt=0  block_type=reinterpret
  reint3 : xbsIndex_r4/Reinterpret  force_arith_type=on  arith_type=Unsigned  force_bin_pt=on  bin_pt=0  block_type=reinterpret
  s_b32a4x1kf_sys0_xeng_pack_out_status_user_data_in : xbsIndex_r4/Gateway Out  inherit_from_input=off  hdl_port=on  rows=1  columns=1  UseAsDAC=off  DACChannel='1'  interface=None  automatic_assignment=on  address_offset=hex2dec('00')  intf_name=''  intf_description=''  timing_constraint=None  locs_specified=off  LOCs={}  io_standard={}  block_type=gatewayout
  sim_out : Terminator
  wires:
  concatenate/1 -> io_delay/1
  io_delay/1 -> cast_gw/1
  cast_gw/1 -> s_b32a4x1kf_sys0_xeng_pack_out_status_user_data_in/1
  s_b32a4x1kf_sys0_xeng_pack_out_status_user_data_in/1 -> sim_out/1
  out_pkt_cnt/1 -> assert_pkt_cnt/1
  assert_pkt_cnt/1 -> reint1/1
  reint1/1 -> concatenate/1
  out_align_err_cnt/1 -> assert_align_err_cnt/1
  assert_align_err_cnt/1 -> reint2/1
  reint2/1 -> concatenate/2
  out_overflow_err_cnt/1 -> assert_overflow_err_cnt/1
  assert_overflow_err_cnt/1 -> reint3/1
  reint3/1 -> concatenate/3

== system s_b16a4x32kf/sys0/xeng_pack_out/vacc_monitor3 ==
  cnt_rst : Inport
  eof : Inport  Port=2
  error : Inport  Port=3
  overflow : Inport  Port=4
  Delay1 : Subsystem  Tag=cmac_delinked  mask(pipeline){csp_latency=2}
      mask prompts: csp_latency "Latency"
      mask help:
      | An explicitly laid-out delay line to avoid mapping to SRL16s
      | for use in pipelining to help achieve timing closure.
      mask init:
      | pipeline_init(gcb,'latency',csp_latency);
      settings: AttributesFormatString=Latency = %<latency>
      mask Display:
      | port_label('input', 1, 'd');
      | port_label('output', 1, 'q');
      | disp(['Z^-', num2str(csp_latency)]);
  Delay2 : Subsystem  Tag=cmac_delinked  mask(pipeline){csp_latency=2}
      mask prompts: csp_latency "Latency"
      mask help:
      | An explicitly laid-out delay line to avoid mapping to SRL16s
      | for use in pipelining to help achieve timing closure.
      mask init:
      | pipeline_init(gcb,'latency',csp_latency);
      settings: AttributesFormatString=Latency = %<latency>
      mask Display:
      | port_label('input', 1, 'd');
      | port_label('output', 1, 'q');
      | disp(['Z^-', num2str(csp_latency)]);
  Delay29 : Subsystem  Tag=cmac_delinked  mask(pipeline){csp_latency=2}
      mask prompts: csp_latency "Latency"
      mask help:
      | An explicitly laid-out delay line to avoid mapping to SRL16s
      | for use in pipelining to help achieve timing closure.
      mask init:
      | pipeline_init(gcb,'latency',csp_latency);
      settings: AttributesFormatString=Latency = %<latency>
      mask Display:
      | port_label('input', 1, 'd');
      | port_label('output', 1, 'q');
      | disp(['Z^-', num2str(csp_latency)]);
  Delay3 : Subsystem  Tag=cmac_delinked  mask(pipeline){csp_latency=2}
      mask prompts: csp_latency "Latency"
      mask help:
      | An explicitly laid-out delay line to avoid mapping to SRL16s
      | for use in pipelining to help achieve timing closure.
      mask init:
      | pipeline_init(gcb,'latency',csp_latency);
      settings: AttributesFormatString=Latency = %<latency>
      mask Display:
      | port_label('input', 1, 'd');
      | port_label('output', 1, 'q');
      | disp(['Z^-', num2str(csp_latency)]);
  Delay4 : Subsystem  Tag=cmac_delinked  mask(pipeline){csp_latency=2}
      mask prompts: csp_latency "Latency"
      mask help:
      | An explicitly laid-out delay line to avoid mapping to SRL16s
      | for use in pipelining to help achieve timing closure.
      mask init:
      | pipeline_init(gcb,'latency',csp_latency);
      settings: AttributesFormatString=Latency = %<latency>
      mask Display:
      | port_label('input', 1, 'd');
      | port_label('output', 1, 'q');
      | disp(['Z^-', num2str(csp_latency)]);
  Delay5 : Subsystem  Tag=cmac_delinked  mask(pipeline){csp_latency=2}
      mask prompts: csp_latency "Latency"
      mask help:
      | An explicitly laid-out delay line to avoid mapping to SRL16s
      | for use in pipelining to help achieve timing closure.
      mask init:
      | pipeline_init(gcb,'latency',csp_latency);
      settings: AttributesFormatString=Latency = %<latency>
      mask Display:
      | port_label('input', 1, 'd');
      | port_label('output', 1, 'q');
      | disp(['Z^-', num2str(csp_latency)]);
  Delay6 : Subsystem  Tag=cmac_delinked  mask(pipeline){csp_latency=2}
      mask prompts: csp_latency "Latency"
      mask help:
      | An explicitly laid-out delay line to avoid mapping to SRL16s
      | for use in pipelining to help achieve timing closure.
      mask init:
      | pipeline_init(gcb,'latency',csp_latency);
      settings: AttributesFormatString=Latency = %<latency>
      mask Display:
      | port_label('input', 1, 'd');
      | port_label('output', 1, 'q');
      | disp(['Z^-', num2str(csp_latency)]);
  payload_cnt1 : xbsIndex_r4/Counter  cnt_type=Free Running  cnt_to=0  operation=Up  start_count=0  cnt_by_val=1  arith_type=Unsigned  n_bits=8  bin_pt=0  load_pin=off  rst=on  en=on  explicit_period=off  period=1  use_behavioral_HDL=on  implementation=Fabric  use_rpm=on  dbl_ovrd=off  block_type=counter
      settings: xl_area=[0, 0, 0, 0, 0, 0, 0]
  payload_cnt2 : xbsIndex_r4/Counter  cnt_type=Free Running  cnt_to=0  operation=Up  start_count=0  cnt_by_val=1  arith_type=Unsigned  n_bits=8  bin_pt=0  load_pin=off  rst=on  en=on  explicit_period=off  period=1  use_behavioral_HDL=on  implementation=Fabric  use_rpm=on  dbl_ovrd=off  block_type=counter
      settings: xl_area=[0, 0, 0, 0, 0, 0, 0]
  payload_cnt3 : xbsIndex_r4/Counter  cnt_type=Free Running  cnt_to=0  operation=Up  start_count=0  cnt_by_val=1  arith_type=Unsigned  n_bits=16  bin_pt=0  load_pin=off  rst=on  en=on  explicit_period=off  period=1  use_behavioral_HDL=on  implementation=Fabric  use_rpm=on  dbl_ovrd=off  block_type=counter
      settings: xl_area=[0, 0, 0, 0, 0, 0, 0]
  pkt_cnt : Outport
  error_cnt : Outport  Port=2
  overflow_cnt : Outport  Port=3
  wires:
  Delay3/1(q) -> pkt_cnt/1
  error/1 -> Delay29/1(d)
  Delay4/1(q) -> error_cnt/1
  eof/1 -> Delay1/1(d)
  cnt_rst/1 -> Delay2/1(d)
  payload_cnt1/1 -> Delay4/1(d)
  Delay29/1(q) -> payload_cnt1/2
  Delay1/1(q) -> payload_cnt3/2
  payload_cnt3/1 -> Delay3/1(d)
  Delay6/1(q) -> overflow_cnt/1
  overflow/1 -> Delay5/1(d)
  Delay5/1(q) -> payload_cnt2/2
  Delay2/1(q) -> payload_cnt1/1, payload_cnt2/1, payload_cnt3/1
  payload_cnt2/1 -> Delay6/1(d)
